simulink model "STEK_roket_simscape_modeli"  (R2025b)
settings: Solver=ode4  StartTime=0.0  StopTime=10.0  FixedStep=0.001  RelTol=1e-3
values from neighbouring files (symbols this model uses):
  m = 0.10*(hi - lo)    [STEK_HIL_grafik_uret.m]
  N = floor(sure_s/TS)    [STEK_HIL_roket_modeli.m]
  s = strrep(sprintf('    [STEK_HIL_grafik_uret.m]
undefined symbols (not defined in the file or in its folder): X, Y, Z
libraries: sm_lib x13, nesl_utility x13, sharedtransform x1
settings Model: SimulationMode=accelerator  Creator=serha  LastModifiedBy=HASAN BARAN

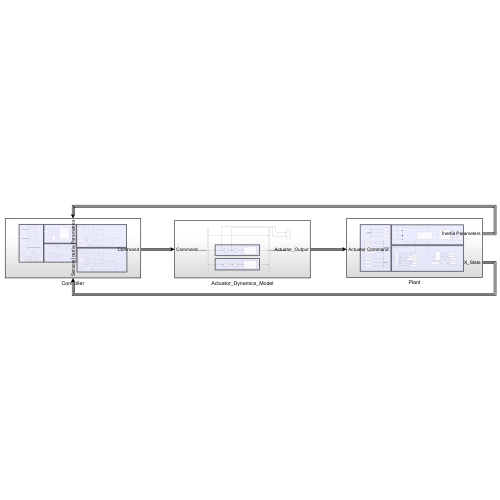
[thumbnail: Simulink's stored preview of the top-level diagram]
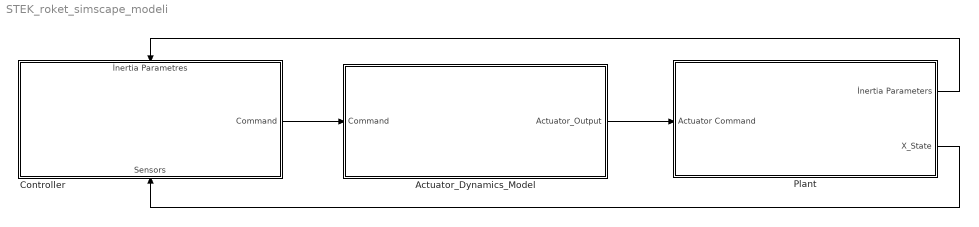
== system STEK_roket_simscape_modeli ==
  Actuator_Dynamics_Model : Subsystem
  Controller : Subsystem
      settings: PortSchema="{\"entries\":[{\"content\":{\"sides\":[{\"content\":{},\"type\":\"ConnectorPlacement.EquallySpacedRectSide\",\"uuid\":\"0baf99d7-4fae-4262-afe2-c6ef4fc7e965\"},{\"content\":{\"connectorIds\":[\"Out1\"],\"side\":\"RIGHT\"},\"type\":\"ConnectorPlacement.EquallySpacedRectSide\",\"uuid\":\"2488a78a-ff3f-460a-aef8-3b0169e54eb5\"},{\"content\":{\"connectorIds\":[\"In1\"],\"side\":\"TOP\"},\"type\":\"ConnectorPlacement.EquallySpacedRectSide\",\"uuid\":\"c1609aa8-bb76-4067-9b78-102063cdf61a\"},{\"content\":{\"connectorIds\":[\"In2\"],\"side\":\"BOTTOM\"},\"type\":\"ConnectorPlacement.EquallySpacedRectSide\",\"uuid\":\"c0f1c736-44b8-4377-a1aa-bd9fc4d2b5f4\"}]},\"type\":\"ConnectorPlacement.EquallySpacedConnector\",\"uuid\":\"1a76828c-b03e-4c12-a774-153e83589147\"}],\"packageUris\":[\"http://schema.mathworks.com/mf0/Connector/R2020b\"],\"version\":\"1.0\"}"
  Plant : Subsystem
  wires:
  Actuator_Dynamics_Model/1(Actuator_Output) -> Plant/1(Actuator Command)
  Controller/1(Command) -> Actuator_Dynamics_Model/1(Command)
  Plant/2(X_State) -> Controller/2(Sensors)
  Plant/1(İnertia Parameters) -> Controller/1(İnertia Parametres)

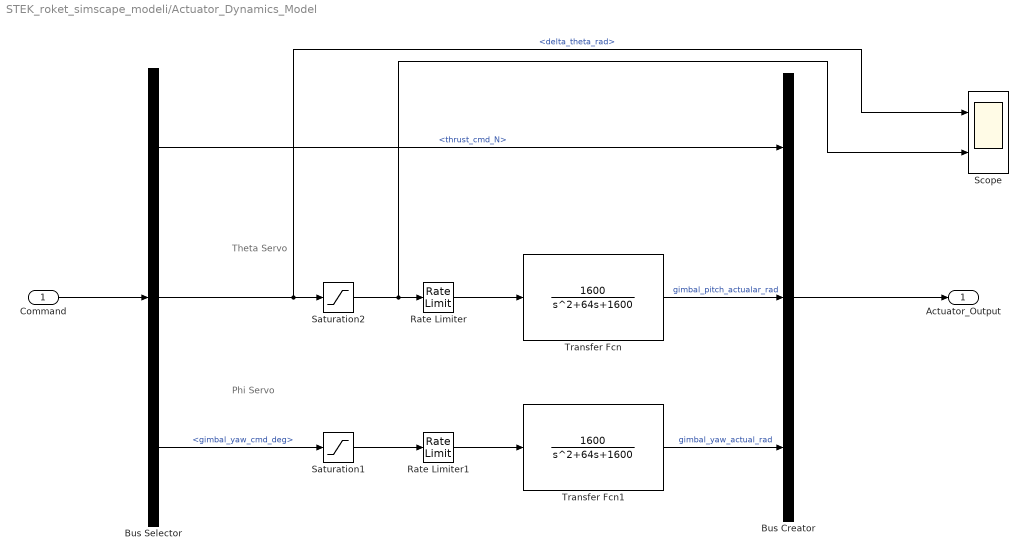
== system STEK_roket_simscape_modeli/Actuator_Dynamics_Model ==
  note: Theta Servo
  note: Phi Servo
  Command : Inport
  Bus Creator : BusCreator  Inputs=3
  Bus Selector : BusSelector  OutputSignals=thrust_cmd_N,delta_theta_rad,gimbal_yaw_cmd_deg
  Rate Limiter : RateLimiter  RisingSlewLimit=428.5  FallingSlewLimit=-428.5  SampleTimeMode=inherited
  Rate Limiter1 : RateLimiter  RisingSlewLimit=428.5  FallingSlewLimit=-428.5  SampleTimeMode=inherited
  Saturation1 : Saturate  UpperLimit=deg2rad(5)  LowerLimit=-deg2rad(5)
  Saturation2 : Saturate  UpperLimit=deg2rad(5)  LowerLimit=-deg2rad(5)
  Scope : Scope  NumInputPorts=2
  Transfer Fcn : TransferFcn  Numerator=1600  Denominator=[1 64 1600]
  Transfer Fcn1 : TransferFcn  Numerator=1600  Denominator=[1 64 1600]
  Actuator_Output : Outport
  wires:
  Command/1 -> Bus Selector/1
  Transfer Fcn/1 -> Bus Creator/2  "gimbal_pitch_actualar_rad"
  Rate Limiter/1 -> Transfer Fcn/1
  Saturation1/1 -> Rate Limiter1/1
  Rate Limiter1/1 -> Transfer Fcn1/1
  Transfer Fcn1/1 -> Bus Creator/3  "gimbal_yaw_actual_rad"
  Bus Selector/3 -> Saturation1/1  "<gimbal_yaw_cmd_deg>"
  Bus Creator/1 -> Actuator_Output/1
  Bus Selector/1 -> Bus Creator/1  "<thrust_cmd_N>"
  Bus Selector/2 -> Scope/1, Saturation2/1  "<delta_theta_rad>"
  Saturation2/1 -> Scope/2, Rate Limiter/1

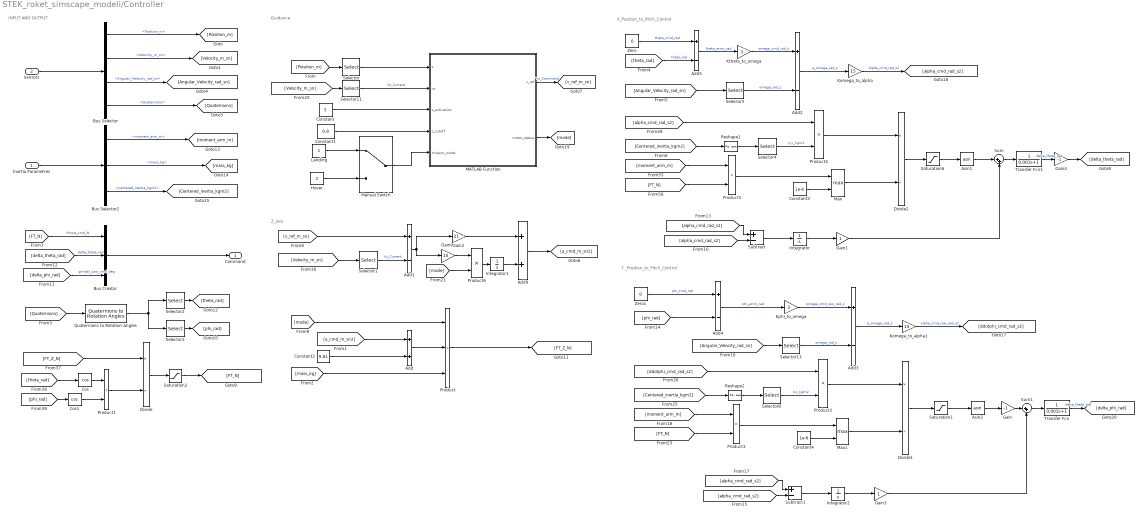
== system STEK_roket_simscape_modeli/Controller ==
  note: Guidance
  note: X_Position_to_Pitch_Control
  note: Z_axis
  note: İNPUT AND OUTPUT
  note: Y _Position_to_Pitch_Control
  İnertia Parametres : Inport
  Sensors : Inport  Port=2
  Add : Sum
  Add{1..5} (5 alike) : Sum  Inputs=+-
  Add9 : Sum
  Asin1 : Trigonometry  Operator=asin
  Asin2 : Trigonometry  Operator=asin
  Bus Creator : BusCreator  Inputs=3
  Bus Selector : BusSelector  OutputSignals=Position_m,Velocity_m_sn,Angular_Velocity_rad_sn,Quaternions
  Bus Selector2 : BusSelector  OutputSignals=moment_arm_m,mass_kg,centered_inertia_kgm2
  Constant : Constant  Value=5
  Constant1 : Constant  Value=0.8
  Constant2 : Constant  Value=9.81
  Constant3 : Constant  Value=1e-6
  Constant4 : Constant  Value=1e-6
  Cos : Trigonometry  Operator=cos
  Cos1 : Trigonometry  Operator=cos
  Divide : Product  Inputs=*/
  Divide1 : Product  Inputs=*/
  Divide2 : Product  Inputs=*/
  Gain : Gain  Gain=-1
  Gain1 : Gain
  Gain2 : Gain  Gain=21
  Gain3 : Gain
  Gain4 : Gain  Gain=-1
  Gain9 : Gain  Gain=15
  Hover : Constant  Value=2
  Integrator : Integrator  LimitOutput=on  UpperSaturationLimit=5  LowerSaturationLimit=-5
  Integrator1 : Integrator  LimitOutput=on  UpperSaturationLimit=7.5  LowerSaturationLimit=-7.5
  Integrator2 : Integrator  LimitOutput=on  UpperSaturationLimit=5  LowerSaturationLimit=-5
  Komega_to_alpha : Gain  Gain=15
  Komega_to_alpha1 : Gain  Gain=15
  Kphi_to_omega : Gain  Gain=3
  Ktheta_to_omega : Gain  Gain=3
  Landing : Constant
  MATLAB Function : MATLAB Function  TreatAsAtomicUnit=on
  Manual Switch : ManualSwitch
  Max : MinMax  Function=max  Inputs=2
  Max1 : MinMax  Function=max  Inputs=2
  Product : Product  Inputs=3
  Product{1..6} (6 alike) : Product
  Quaternions to Rotation Angles : sharedtransform/Quaternions to Rotation Angles  rotationOrder=ZYX  aMode=aMode
  Reshape1 : Reshape
  Reshape2 : Reshape
  Saturation1 : Saturate  UpperLimit=1  LowerLimit=-1
  Saturation2 : Saturate  UpperLimit=600  LowerLimit=0
  Saturation6 : Saturate  UpperLimit=1  LowerLimit=-1
  Selector{,1,3,11,13} (5 alike) : Selector  InputPortWidth=3  IndexOptions=Index vector (dialog)  Indices=3  OutputSizes=1
  Selector2 : Selector  InputPortWidth=3  IndexOptions=Index vector (dialog)  Indices=2  OutputSizes=1
  Selector4 : Selector  InputPortWidth=9  IndexOptions=Index vector (dialog)  Indices=5  OutputSizes=1
  Selector5 : Selector  InputPortWidth=3  IndexOptions=Index vector (dialog)  Indices=2  OutputSizes=1
  Selector8 : Selector  InputPortWidth=9  IndexOptions=Index vector (dialog)  Indices=1  OutputSizes=1
  Subtract : Sum  Inputs=+-
  Subtract1 : Sum  Inputs=+-
  Sum : Sum  Inputs=|++
  Sum1 : Sum  Inputs=|++
  Transfer Fcn : TransferFcn  Denominator=[0.001 1]
  Transfer Fcn1 : TransferFcn  Denominator=[0.001 1]
  Zero : Constant  Value=0  OutDataTypeStr=Inherit: Inherit via back propagation
  Zero1 : Constant  Value=0  OutDataTypeStr=Inherit: Inherit via back propagation
  Command : Outport
  wires:
  Sensors/1 -> Bus Selector/1
  Bus Selector2/2 -> [mass_kg]  "<mass_kg>"
  İnertia Parametres/1 -> Bus Selector2/1
  Bus Selector2/1 -> [moment_arm_m]  "<moment_arm_m>"
  Bus Selector2/3 -> [Centered_inertia_kgm2]  "<centered_inertia_kgm2>"
  Bus Creator/1 -> Command/1
  [delta_phi_rad] -> Bus Creator/3  "gimbal_yaw_cmd_deg"
  [FT_N] -> Bus Creator/1  "thrust_cmd_N"
  [delta_theta_rad] -> Bus Creator/2  "delta_theta_rad"
  [Velocity_m_sn] -> Selector1/1
  Gain2/1 -> Add9/1
  Add1/1 -> Gain9/1, Gain2/1
  Integrator1/1 -> Add9/2
  Selector1/1 -> Add1/2  "Vz_Current"
  Constant2/1 -> Add/2
  [a_cmd_m_sn2] -> Add/1
  Add/1 -> Product/2
  [mass_kg] -> Product/3
  Product/1 -> [FT_Z_N]
  Reshape1/1 -> Selector4/1
  Add5/1 -> Ktheta_to_omega/1  "theta_error_rad"
  Divide2/1 -> Saturation6/1
  [Centered_inertia_kgm2] -> Reshape1/1
  Selector4/1 -> Product4/2  "Iyy_kgm2"
  Sum/1 -> Transfer Fcn1/1
  Product4/1 -> Divide2/1
  Transfer Fcn1/1 -> Gain4/1  "delta_theta_rad"
  Asin1/1 -> Sum/1
  Product5/1 -> Max/1
  [alpha_cmd_rad_s2] -> Product4/1
  [moment_arm_m] -> Product5/1
  [FT_N] -> Product5/2
  Add2/1 -> Komega_to_alpha/1  "e_omega_rad_s"
  Ktheta_to_omega/1 -> Add2/1  "omega_cmd_rad_s"
  [Quaternions] -> Quaternions to Rotation Angles/1
  Quaternions to Rotation Angles/1 -> Selector3/1, Selector2/1
  Selector3/1 -> [phi_rad]
  Selector2/1 -> [theta_rad]
  [Angular_Velocity_rad_sn] -> Selector5/1
  Product1/1 -> Divide/2
  [FT_Z_N] -> Divide/1
  Divide/1 -> Saturation2/1
  Cos1/1 -> Product1/2
  Cos/1 -> Product1/1
  [phi_rad] -> Cos1/1
  [theta_rad] -> Cos/1
  [theta_rad] -> Add5/2  "theta_rad"
  Selector5/1 -> Add2/2  "omega_rad_s"
  [v_ref_m_sn] -> Add1/1
  [mode] -> Product/1
  Max/1 -> Divide2/2
  Constant3/1 -> Max/2
  Saturation6/1 -> Asin1/1
  [mode] -> Product6/2
  Add9/1 -> [a_cmd_m_sn2]
  Gain9/1 -> Product6/1
  Komega_to_alpha/1 -> [alpha_cmd_rad_s2]  "alpha_cmd_rad_s2"
  Saturation1/1 -> Asin2/1
  Constant4/1 -> Max1/2
  Max1/1 -> Divide1/2
  Selector13/1 -> Add3/2  "omega_rad_s"
  [phi_rad] -> Add4/2
  [Angular_Velocity_rad_sn] -> Selector13/1
  Komega_to_alpha1/1 -> [ddotphi_cmd_rad_s2]  "alpha_cmd_raw_rad_s2"
  Kphi_to_omega/1 -> Add3/1  "omega_cmd_raw_rad_s"
  Add3/1 -> Komega_to_alpha1/1  "e_omega_rad_s"
  [FT_N] -> Product3/2
  [moment_arm_m] -> Product3/1
  [ddotphi_cmd_rad_s2] -> Product2/1
  Product3/1 -> Max1/1
  Transfer Fcn/1 -> [delta_phi_rad]  "delta_theta_rad"
  Product2/1 -> Divide1/1
  Selector8/1 -> Product2/2  "Ixx_kgm2"
  [Centered_inertia_kgm2] -> Reshape2/1
  Divide1/1 -> Saturation1/1
  Add4/1 -> Kphi_to_omega/1  "phi_error_rad"
  Reshape2/1 -> Selector8/1
  Asin2/1 -> Gain/1
  Zero/1 -> Add5/1  "theta_cmd_rad"
  Zero1/1 -> Add4/1  "phi_cmd_rad"
  Gain/1 -> Sum1/1
  Bus Selector/3 -> [Angular_Velocity_rad_sn]  "<Angular_Velocity_rad_sn>"
  Bus Selector/2 -> [Velocity_m_sn]  "<Velocity_m_sn>"
  Bus Selector/4 -> [Quaternions]  "<Quaternions>"
  Bus Selector/1 -> [Poisition_m]  "<Position_m>"
  Constant/1 -> MATLAB Function/3(z_activation)
  MATLAB Function/2(motor_status) -> [mode]
  [Poisition_m] -> Selector/1
  Constant1/1 -> MATLAB Function/4(z_cutoff)
  Selector/1 -> MATLAB Function/1(z)
  Selector11/1 -> MATLAB Function/2(vz)  "Vz_Current"
  MATLAB Function/1(v_ref) -> [v_ref_m_sn]  "Vz_Command"
  [Velocity_m_sn] -> Selector11/1
  Saturation2/1 -> [FT_N]
  Product6/1 -> Integrator1/1
  Manual Switch/1 -> MATLAB Function/5(mission_mode)
  Hover/1 -> Manual Switch/2
  Landing/1 -> Manual Switch/1
  [alpha_cmd_rad_s2] -> Subtract/1
  Integrator/1 -> Gain1/1
  Subtract/1 -> Integrator/1
  [alpha_cmd_rad_s2] -> Subtract/2
  Gain1/1 -> Sum/2
  [alpha_cmd_rad_s2] -> Subtract1/2
  Integrator2/1 -> Gain3/1
  Gain3/1 -> Sum1/2
  Subtract1/1 -> Integrator2/1
  [alpha_cmd_rad_s2] -> Subtract1/1
  Sum1/1 -> Transfer Fcn/1
  Gain4/1 -> [delta_theta_rad]

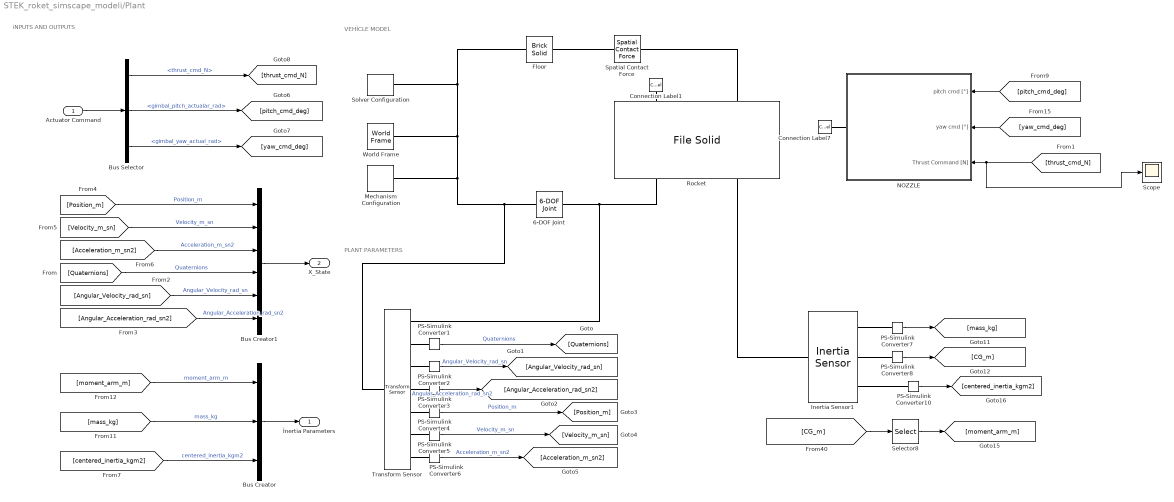
== system STEK_roket_simscape_modeli/Plant ==
  note: VEHİCLE MODEL
  note: iNPUTS AND OUTPUTS
  note: PLANT PARAMETERS
  Actuator Command : Inport
  6-DOF Joint : sm_lib/Joints/6-DOF Joint  JointMode=Normal  CompositeWrenchDir=FollowerOnBase  CompositeWrenchFrame=BaseFrame  SenseConstraintForce=off  SenseConstraintTorque=off  SenseTotalForce=off  SenseTotalTorque=off  PxPositionTargetSpecify=off  PxPositionTargetPriority=High  PxPositionTargetValue=0  PxPositionTargetValueUnits=m  PxVelocityTargetSpecify=off  PxVelocityTargetPriority=High  PxVelocityTargetValue=0  PxVelocityTargetValueUnits=m/s  PxEquilibriumPosition=0  PxEquilibriumPositionUnits=m  PxSpringStiffness=0  PxSpringStiffnessUnits=N/m  PxDampingCoefficient=0  PxDampingCoefficientUnits=N/(m/s)  PxLowerLimitSpecify=off  PxLowerLimitBound=-1  PxLowerLimitBoundUnits=m  PxLowerLimitStiffness=1e6  PxLowerLimitStiffnessUnits=N/m  PxLowerLimitDamping=1e3  PxLowerLimitDampingUnits=N/(m/s)  PxLowerLimitTransitionRegionWidth=1e-4  PxLowerLimitTransitionRegionWidthUnits=m  PxUpperLimitSpecify=off  PxUpperLimitBound=1  PxUpperLimitBoundUnits=m  PxUpperLimitStiffness=1e6  PxUpperLimitStiffnessUnits=N/m  PxUpperLimitDamping=1e3  PxUpperLimitDampingUnits=N/(m/s)  PxUpperLimitTransitionRegionWidth=1e-4  PxUpperLimitTransitionRegionWidthUnits=m  PxTorqueActuationMode=NoTorque  PxMotionActuationMode=ComputedMotion  PxSensePosition=off  PxSenseVelocity=off  PxSenseAcceleration=off  PxSenseTorqueForce=off  PxSenseLowerLimitTorqueForce=off  PxSenseUpperLimitTorqueForce=off  PyPositionTargetSpecify=off  PyPositionTargetPriority=High  PyPositionTargetValue=0  PyPositionTargetValueUnits=m  PyVelocityTargetSpecify=off  PyVelocityTargetPriority=High  PyVelocityTargetValue=0  PyVelocityTargetValueUnits=m/s  PyEquilibriumPosition=0  PyEquilibriumPositionUnits=m  PySpringStiffness=0  PySpringStiffnessUnits=N/m  PyDampingCoefficient=0  PyDampingCoefficientUnits=N/(m/s)  PyLowerLimitSpecify=off  PyLowerLimitBound=-1  PyLowerLimitBoundUnits=m  PyLowerLimitStiffness=1e6  PyLowerLimitStiffnessUnits=N/m  PyLowerLimitDamping=1e3  PyLowerLimitDampingUnits=N/(m/s)  PyLowerLimitTransitionRegionWidth=1e-4  PyLowerLimitTransitionRegionWidthUnits=m  PyUpperLimitSpecify=off  PyUpperLimitBound=1  PyUpperLimitBoundUnits=m  PyUpperLimitStiffness=1e6  PyUpperLimitStiffnessUnits=N/m  PyUpperLimitDamping=1e3  PyUpperLimitDampingUnits=N/(m/s)  PyUpperLimitTransitionRegionWidth=1e-4  PyUpperLimitTransitionRegionWidthUnits=m  PyTorqueActuationMode=NoTorque  PyMotionActuationMode=ComputedMotion  PySensePosition=off  PySenseVelocity=off  PySenseAcceleration=off  PySenseTorqueForce=off  PySenseLowerLimitTorqueForce=off  PySenseUpperLimitTorqueForce=off  PzPositionTargetSpecify=on  PzPositionTargetPriority=High  PzPositionTargetValue=8  PzPositionTargetValueUnits=m  PzVelocityTargetSpecify=off  PzVelocityTargetPriority=High  PzVelocityTargetValue=0  PzVelocityTargetValueUnits=m/s  PzEquilibriumPosition=0  PzEquilibriumPositionUnits=m  PzSpringStiffness=0  PzSpringStiffnessUnits=N/m  PzDampingCoefficient=0  PzDampingCoefficientUnits=N/(m/s)  PzLowerLimitSpecify=off  PzLowerLimitBound=-1  PzLowerLimitBoundUnits=m  PzLowerLimitStiffness=1e6  PzLowerLimitStiffnessUnits=N/m  PzLowerLimitDamping=1e3  PzLowerLimitDampingUnits=N/(m/s)  PzLowerLimitTransitionRegionWidth=1e-4  PzLowerLimitTransitionRegionWidthUnits=m  PzUpperLimitSpecify=off  PzUpperLimitBound=1  PzUpperLimitBoundUnits=m  PzUpperLimitStiffness=1e6  PzUpperLimitStiffnessUnits=N/m  PzUpperLimitDamping=1e3  PzUpperLimitDampingUnits=N/(m/s)  PzUpperLimitTransitionRegionWidth=1e-4  PzUpperLimitTransitionRegionWidthUnits=m  PzTorqueActuationMode=NoTorque  PzMotionActuationMode=ComputedMotion  PzSensePosition=off  PzSenseVelocity=off  PzSenseAcceleration=off  PzSenseTorqueForce=off  PzSenseLowerLimitTorqueForce=off  PzSenseUpperLimitTorqueForce=off  SphPositionTargetSpecify=off  SphPositionTargetPriority=High  SphPositionTargetRotationMethod=StandardAxis  SphPositionTargetFollAlignAxisA=+X  SphPositionTargetBaseAlignAxisA=+Y  SphPositionTargetFollAlignAxisB=+Y  SphPositionTargetBaseAlignAxisB=+Z  SphPositionTargetRotationStandardAxis=+X  SphPositionTargetRotationAngle=5  SphPositionTargetRotationAngleUnits=deg  SphPositionTargetRotationArbitraryAxis=[0 0 1]  SphPositionTargetRotationSequenceAxes=FollowerAxes  SphPositionTargetRotationSequence=ZYX  SphPositionTargetRotationSequenceAngles=[0 0 0]  SphPositionTargetRotationSequenceAnglesUnits=deg  SphPositionTargetRotationMatrix=[1 0 0;0 1 0;0 0 1]  SphPositionTargetQuaternion=[1 0 0 0]  SphVelocityTargetSpecify=off  SphVelocityTargetPriority=High  SphVelocityTargetValue=[0 0 0]  SphVelocityTargetValueUnits=deg/s  SphVelocityTargetInFollowerFrame=on  SphEqPosRotationMethod=None  SphEqPosFollAlignAxisA=+X  SphEqPosBaseAlignAxisA=+Y  SphEqPosFollAlignAxisB=+Y  SphEqPosBaseAlignAxisB=+Z  SphEqPosRotationStandardAxis=+Z  SphEqPosRotationAngle=0  SphEqPosRotationAngleUnits=deg  SphEqPosRotationArbitraryAxis=[0 0 1]  SphEqPosRotationSequenceAxes=FollowerAxes  SphEqPosRotationSequence=XYX  SphEqPosRotationSequenceAngles=[0 0 0]  SphEqPosRotationSequenceAnglesUnits=deg  SphEqPosRotationMatrix=[1 0 0;0 1 0;0 0 1]  SphEqPosQuaternion=[1 0 0 0]  SphSpringStiffness=0  SphSpringStiffnessUnits=N*m/deg  SphDampingCoefficient=0  SphDampingCoefficientUnits=N*m/(deg/s)  SphLowerLimitSpecify=off  SphLowerLimitBound=15  SphLowerLimitBoundUnits=deg  SphLowerLimitStiffness=1e4  SphLowerLimitStiffnessUnits=N*m/deg  SphLowerLimitDamping=10  SphLowerLimitDampingUnits=N*m/(deg/s)  SphLowerLimitTransitionRegionWidth=0.1  SphLowerLimitTransitionRegionWidthUnits=deg  SphUpperLimitSpecify=off  SphUpperLimitBound=45  SphUpperLimitBoundUnits=deg  SphUpperLimitStiffness=1e4  SphUpperLimitStiffnessUnits=N*m/deg  SphUpperLimitDamping=10  SphUpperLimitDampingUnits=N*m/(deg/s)  SphUpperLimitTransitionRegionWidth=0.1  SphUpperLimitTransitionRegionWidthUnits=deg  SphTorqueActuationMode=NoTorque  SphActuateTorqueX=off  SphActuateTorqueY=off  SphActuateTorqueZ=off  SphActuateTorque=off  SphActuationFrame=BaseFrame  SphSensePosition=off  SphSenseVelocityX=off  SphSenseVelocityY=off  SphSenseVelocityZ=off  SphSenseVelocity=off  SphSenseAccelerationX=off  SphSenseAccelerationY=off  SphSenseAccelerationZ=off  SphSenseAcceleration=off  SphSenseLowerLimitTorqueMag=off  SphSenseUpperLimitTorqueMag=off  SphSensingFrame=BaseFrame
  Bus Creator : BusCreator  Inputs=3
  Bus Creator1 : BusCreator  Inputs=6
  Bus Selector : BusSelector  OutputSignals=thrust_cmd_N,gimbal_pitch_actualar_rad,gimbal_yaw_actual_rad
  Connection Label1 : ConnectionLabel  Label=NOZZLE
  Connection Label7 : ConnectionLabel  Label=NOZZLE
  Floor : sm_lib/Body Elements/Brick Solid  BrickDimensions=[5 5 0.5]  BrickDimensionsUnits=m  ExportEntireGeometry=on  InertiaType=CalculateFromGeometry  BasedOnType=Density  Density=0  DensityUnits=kg/m^3  Mass=1  MassUnits=kg  CenterOfMass=[0 0 0]  CenterOfMassUnits=m  MomentsOfInertia=[1 1 1]  MomentsOfInertiaUnits=kg*m^2  ProductsOfInertia=[0 0 0]  ProductsOfInertiaUnits=kg*m^2  GraphicType=FromGeometry  MarkerShape=Sphere  MarkerSize=10  GraphicVisPropType=SimpleVisualProperties  GraphicDiffuseColor=[1 0.6667 0]  GraphicOpacity=1  GraphicSpecularColor=[0.5 0.5 0.5 1.0]  GraphicAmbientColor=[0.15 0.15 0.15 1.0]  GraphicEmissiveColor=[0.0 0.0 0.0 1.0]  GraphicShininess=75  DoExposeReferenceFrame=on  SerializedFrames=<Frames/>
  Inertia Sensor1 : sm_lib/Body Elements/Inertia Sensor  SensorExtent=Mechanism  SpanWeldJoints=off  ExcludeGroundedBodies=off  MeasurementFrame=Attached  SenseMass=on  SenseCenterOfMass=on  SenseInertiaMatrix=off  SenseCenteredInertiaMatrix=on  SensePrincipalInertiaMatrix=off  SenseRotationMatrix=off  GraphicType=PrincipalInertiaFrame  PrincipalInertiaFrameSize=20  GraphicVisPropType=SimpleVisualProperties  GraphicDiffuseColor=[0.5 0.5 0.5]  GraphicOpacity=1  GraphicSpecularColor=[0.5 0.5 0.5 1.0]  GraphicAmbientColor=[0.15 0.15 0.15 1.0]  GraphicEmissiveColor=[0.0 0.0 0.0 1.0]  GraphicShininess=75
  Mechanism Configuration : sm_lib/Utilities/Mechanism Configuration  UniformGravity=Constant  GravityVector=[0 0 -9.80665]  GravityVectorUnits=m/s^2  LinearizationDelta=0.001  JointModeTransitionNonlinearIterations=2
  NOZZLE : Subsystem
  PS-Simulink Converter{1..8,10} (9 alike) : nesl_utility/PS-Simulink Converter  PhysicalDomain=network_engine_domain  SubClassName=ps_output  LeftPortType=input  RightPortType=output  PseudoPeriodic=off  Frequencies=[]  VectorFormat=inherit  Unit=inherit  AffineConversion=off
  Rocket : sm_lib/Body Elements/File Solid  ExtGeomFileName=C:\Users\HASAN BARAN\Desktop\Stek ahr\AHR CAD DOSYALARI\Tvc yok koordinat.STEP  UnitType=Custom  ExtGeomFileUnits=mm  StepReaderType=HEX  ExportConvexHullGeometry=on  InertiaType=CalculateFromGeometry  BasedOnType=Mass  Density=1000  DensityUnits=kg/m^3  Mass=32  MassUnits=kg  CenterOfMass=[0 0 0]  CenterOfMassUnits=m  MomentsOfInertia=[1 1 1]  MomentsOfInertiaUnits=kg*m^2  ProductsOfInertia=[0 0 0]  ProductsOfInertiaUnits=kg*m^2  GraphicType=FromGeometry  MarkerShape=Sphere  MarkerSize=10  GraphicVisPropType=SimpleVisualProperties  GraphicDiffuseColor=[0.5 0.5 0.5]  GraphicOpacity=1  GraphicSpecularColor=[0.5 0.5 0.5 1.0]  GraphicAmbientColor=[0.15 0.15 0.15 1.0]  GraphicEmissiveColor=[0.0 0.0 0.0 1.0]  GraphicShininess=75  DoExposeReferenceFrame=off  SerializedFrames=<Frames><Frame><Id>Frame1</Id><Value><Name>CoM</Name><Origin><Source>CenterOfMassFrame</Source><FeatureName></FeatureName></Origin><PrimaryAxis><DefinedDirection>+Z</DefinedDirection><Source>ReferenceFrame</Source><SourceDirection>+Z</SourceDirection><FeatureName></FeatureName></PrimaryAxis><SecondaryAxis><DefinedDirection>+X</DefinedDirection><Source>ReferenceFrame</Source><SourceDirection>+X</SourceDirection><FeatureName></FeatureName></SecondaryAxis></Value></Frame><Frame><Id>Frame2</Id><Value><Name>TVC</Name><Origin><Source>GeometricFeature</Source><FeatureName>planar surface 130</FeatureName></Origin><PrimaryAxis><DefinedDirection>+Z</DefinedDirection><Source>ReferenceFrame</Source><SourceDirection>+X</SourceDirection><FeatureName></FeatureName></PrimaryAxis><SecondaryAxis><DefinedDirection>+X</DefinedDirection><Source>ReferenceFrame</Source><SourceDirection>-Z</SourceDirection><FeatureName></FeatureName></SecondaryAxis></Value></Frame><Frame><Id>Frame3</Id><Value><Name>İnertia_Sensor</Name><Origin><Source>GeometricFeature</Source><FeatureName>planar surface 130</FeatureName></Origin><PrimaryAxis><DefinedDirection>+Z</DefinedDirection><Source>ReferenceFrame</Source><SourceDirection>+Z</SourceDirection><FeatureName></FeatureName></PrimaryAxis><SecondaryAxis><DefinedDirection>+X</DefinedDirection><Source>ReferenceFrame</Source><SourceDirection>+X</SourceDirection><FeatureName></FeatureName></SecondaryAxis></Value></Frame></Frames>
  Scope : Scope
      settings: ActiveDisplayYMinimum=-1  ActiveDisplayYMaximum=1
  Selector8 : Selector  InputPortWidth=3  IndexOptions=Index vector (dialog)  Indices=3  OutputSizes=1
  Solver Configuration : nesl_utility/Solver Configuration  PhysicalDomain=network_engine_domain  SubClassName=solver  LeftPortType=input  RightPortType=generic  Tones=[]  Harmonics=[]  SimulateNoise=off  Profile=off  UseLocalSampling=off  EnableSwitchedLinearOptims=on  FrequencyDomain=off  UseCCode=off  RelTol=0.001  AbsTol=1e-06  MinStep=1e-09  ToWorkspace=off  RevertToSquareIcSolve=off  NumHomotopyIterations=100  PhasorMode=off  PhasorModeNumHarmonics=1  ConsistencySolver=NEWTON_XTOL_AFTER_FTOL  IndexReductionMethod=DerivativeReplacement  DoDC=off  ResidualTolerance=1e-09  ConsistencyTolSource=GLOBAL  ConsistencyAbsTol=0.001  ConsistencyRelTol=0.001  ConsistencyTolFactor=0.001  UseLocalSolver=off  LocalSolverChoice=NE_BACKWARD_EULER_ADVANCER  ResolveIndetEquations=on  FunctionEvalNumThread=1  LocalSolverSampleTime=0.001  DoFixedCost=off  MaxNonlinIter=3  MaxModeIter=2  ComputeImpulses=off  ImpulseIterations=2  LinearAlgebra=Sparse  LinearAlgebraNumThread=0  EquationFormulation=NE_TIME_EF  DelaysMemoryBudget=1024  AutomaticFiltering=on  FilteringTimeConstant=0.001  PartitionStorageMethod=AS_NEEDED  PartitionMemoryBudget=1024  PartitionMethod=FAST  MultibodyUseLocalSolver=off  MultibodyLocalSolverChoice=ODE1  MultibodyLocalSolverSampleTime=0.001
  Spatial Contact Force : sm_lib/Forces and Torques/Spatial Contact Force  SenseSeparationDistance=off  NormalForceType=SmoothSpringDamper  NormalStiffness=1e6  NormalStiffnessUnits=N/m  NormalDamping=1e3  NormalDampingUnits=N/(m/s)  NormalTransitionRegionWidth=1e-4  NormalTransitionRegionWidthUnits=m  FrictionType=SmoothStickSlip  CoefficientOfStaticFriction=0.5  CoefficientOfDynamicFriction=0.3  FrictionalCriticalVelocity=1e-3  FrictionalCriticalVelocityUnits=m/s  SenseContactSignal=off  SensePenetrationDepth=off  SenseNormalVelocity=off  SenseTangentialVelocity=off  SensingForceTorqueDirection=BaseOnFollower  SensingForceTorqueResolutionFrame=ContactFrame  SenseNormalForce=off  SenseNormalForceMagnitude=off  SenseNormalTorque=off  SenseFrictionalForce=off  SenseFrictionalForceMagnitude=off  SenseFrictionalTorque=off  SenseTotalForce=off  SenseTotalTorque=off  SenseContactBaseRotation=off  SenseContactBaseTranslation=off  SenseContactFollowerRotation=off  SenseContactFollowerTranslation=off  ZeroCrossDetectContactStartAndEnd=off
  Transform Sensor : sm_lib/Frames and Transforms/Transform Sensor  MeasurementFrame=World  RotationSequence=ZYX  SenseAngle=off  SenseAxis=off  SenseQ=on  SenseR=off  SenseRotationSequence=off  SenseOmegaX=off  SenseOmegaY=off  SenseOmegaZ=off  SenseOmega=on  SenseQDot=off  SenseRDot=off  SenseRotationSequenceDot=off  SenseAlphaX=off  SenseAlphaY=off  SenseAlphaZ=off  SenseAlpha=on  SenseQDDot=off  SenseRDDot=off  SenseX=off  SenseY=off  SenseZ=off  SenseXYZ=on  SenseRad=off  SenseAzim=off  SenseDist=off  SenseInc=off  SenseXDot=off  SenseYDot=off  SenseZDot=off  SenseXYZDot=on  SenseRadDot=off  SenseAzimDot=off  SenseDistDot=off  SenseIncDot=off  SenseXDDot=off  SenseYDDot=off  SenseZDDot=off  SenseXYZDDot=on  SenseRadDDot=off  SenseAzimDDot=off  SenseDistDDot=off  SenseIncDDot=off
  World Frame : sm_lib/Frames and Transforms/World Frame
  İnertia Parameters : Outport
  X_State : Outport  Port=2
  wires:
  Bus Creator1/1 -> X_State/1
  Actuator Command/1 -> Bus Selector/1
  [Position_m] -> Bus Creator1/1  "Position_m"
  PS-Simulink Converter7/1 -> [mass_kg]
  [Quaternions] -> Bus Creator1/4  "Quaternions"
  Bus Selector/3 -> [yaw_cmd_deg]  "<gimbal_yaw_actual_rad>"
  [centered_inertia_kgm2] -> Bus Creator/3  "centered_inertia_kgm2"
  Bus Creator/1 -> İnertia Parameters/1
  [Velocity_m_sn] -> Bus Creator1/2  "Velocity_m_sn"
  PS-Simulink Converter3/1 -> [Angular_Acceleration_rad_sn2]  "Angular_Acceleration_rad_sn2"
  [Angular_Acceleration_rad_sn2] -> Bus Creator1/6  "Angular_Acceleration_rad_sn2"
  [Acceleration_m_sn2] -> Bus Creator1/3  "Acceleration_m_sn2"
  Selector8/1 -> [moment_arm_m]
  PS-Simulink Converter8/1 -> [CG_m]
  [moment_arm_m] -> Bus Creator/1  "moment_arm_m"
  PS-Simulink Converter1/1 -> [Quaternions]  "Quaternions"
  [mass_kg] -> Bus Creator/2  "mass_kg"
  [CG_m] -> Selector8/1
  PS-Simulink Converter6/1 -> [Acceleration_m_sn2]  "Acceleration_m_sn2"
  PS-Simulink Converter5/1 -> [Velocity_m_sn]  "Velocity_m_sn"
  PS-Simulink Converter2/1 -> [Angular_Velocity_rad_sn]  "Angular_Velocity_rad_sn"
  Bus Selector/2 -> [pitch_cmd_deg]  "<gimbal_pitch_actualar_rad>"
  PS-Simulink Converter10/1 -> [centered_inertia_kgm2]
  PS-Simulink Converter4/1 -> [Position_m]  "Position_m"
  [Angular_Velocity_rad_sn] -> Bus Creator1/5  "Angular_Velocity_rad_sn"
  [yaw_cmd_deg] -> NOZZLE/2(yaw cmd [°])
  [pitch_cmd_deg] -> NOZZLE/1(pitch cmd [°])
  [thrust_cmd_N] -> Scope/1, NOZZLE/3(Thrust Command [N])
  Bus Selector/1 -> [thrust_cmd_N]  "<thrust_cmd_N>"
  connections:
  World Frame/RConn1 -- Floor/RConn1 -- Solver Configuration/RConn1 -- Transform Sensor/LConn1 -- 6-DOF Joint/LConn1 -- Mechanism Configuration/RConn1
  Rocket/LConn1 -- 6-DOF Joint/RConn1 -- Transform Sensor/RConn1
  Connection Label1/LConn1 -- Rocket/RConn1
  Floor/LConn1 -- Spatial Contact Force/LConn1
  Inertia Sensor1/RConn3 -- PS-Simulink Converter10/LConn1
  NOZZLE/RConn1 -- Connection Label7/LConn1
  Transform Sensor/RConn6 -- PS-Simulink Converter5/LConn1
  PS-Simulink Converter7/LConn1 -- Inertia Sensor1/RConn1
  Transform Sensor/RConn7 -- PS-Simulink Converter6/LConn1
  PS-Simulink Converter3/LConn1 -- Transform Sensor/RConn4
  Rocket/RConn2 -- Spatial Contact Force/RConn1
  PS-Simulink Converter4/LConn1 -- Transform Sensor/RConn5
  PS-Simulink Converter1/LConn1 -- Transform Sensor/RConn2
  PS-Simulink Converter2/LConn1 -- Transform Sensor/RConn3
  Inertia Sensor1/RConn2 -- PS-Simulink Converter8/LConn1
  Rocket/LConn2 -- Inertia Sensor1/LConn1

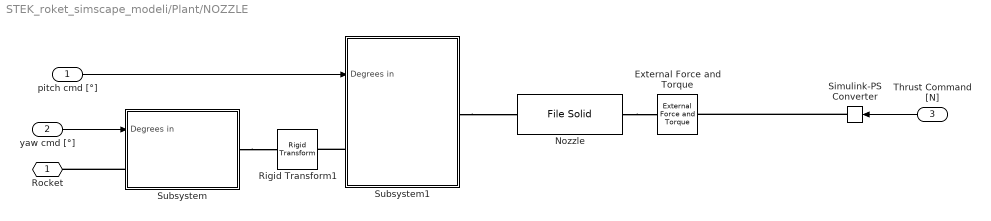
== system STEK_roket_simscape_modeli/Plant/NOZZLE ==
  pitch cmd [°] : Inport
  yaw cmd [°] : Inport  Port=2
  Thrust Command [N] : Inport  Port=3
  External Force and Torque : sm_lib/Forces and Torques/External Force and Torque  EnableForceX=off  EnableForceY=off  EnableForceZ=on  EnableForce=off  ForceResolutionFrame=AttachedFrame  EnableTorqueX=off  EnableTorqueY=off  EnableTorqueZ=off  EnableTorque=off  TorqueResolutionFrame=AttachedFrame
  Nozzle : sm_lib/Body Elements/File Solid  ExtGeomFileName=C:\Users\HASAN BARAN\Desktop\Stek ahr\AHR CAD DOSYALARI\Tvc montaj koordinat.STEP  UnitType=FromFile  ExtGeomFileUnits=m  StepReaderType=HEX  ExportConvexHullGeometry=off  InertiaType=CalculateFromGeometry  BasedOnType=Mass  Density=1000  DensityUnits=kg/m^3  Mass=1.8  MassUnits=kg  CenterOfMass=[0 0 0]  CenterOfMassUnits=m  MomentsOfInertia=[1 1 1]  MomentsOfInertiaUnits=kg*m^2  ProductsOfInertia=[0 0 0]  ProductsOfInertiaUnits=kg*m^2  GraphicType=FromGeometry  MarkerShape=Sphere  MarkerSize=10  GraphicVisPropType=SimpleVisualProperties  GraphicDiffuseColor=[0.5 0.5 0.5]  GraphicOpacity=1  GraphicSpecularColor=[0.5 0.5 0.5 1.0]  GraphicAmbientColor=[0.15 0.15 0.15 1.0]  GraphicEmissiveColor=[0.0 0.0 0.0 1.0]  GraphicShininess=75  DoExposeReferenceFrame=off  SerializedFrames=<Frames><Frame><Id>Frame1</Id><Value><Name>Rocket</Name><Origin><Source>GeometricFeature</Source><FeatureName>planar surface 43</FeatureName></Origin><PrimaryAxis><DefinedDirection>+Z</DefinedDirection><Source>ReferenceFrame</Source><SourceDirection>+Y</SourceDirection><FeatureName></FeatureName></PrimaryAxis><SecondaryAxis><DefinedDirection>-Y</DefinedDirection><Source>ReferenceFrame</Source><SourceDirection>+X</SourceDirection><FeatureName></FeatureName></SecondaryAxis></Value></Frame><Frame><Id>Frame2</Id><Value><Name>Thrust</Name><Origin><Source>GeometricFeature</Source><FeatureName>planar surface 44</FeatureName></Origin><PrimaryAxis><DefinedDirection>+Z</DefinedDirection><Source>ReferenceFrame</Source><SourceDirection>+Z</SourceDirection><FeatureName></FeatureName></PrimaryAxis><SecondaryAxis><DefinedDirection>+X</DefinedDirection><Source>ReferenceFrame</Source><SourceDirection>+X</SourceDirection><FeatureName></FeatureName></SecondaryAxis></Value></Frame></Frames>
  Rigid Transform1 : sm_lib/Frames and Transforms/Rigid Transform  RotationMethod=StandardAxis  FollAlignAxisA=+X  BaseAlignAxisA=+Y  FollAlignAxisB=+Y  BaseAlignAxisB=+Z  RotationStandardAxis=+X  RotationAngle=-90  RotationAngleUnits=deg  RotationArbitraryAxis=[0 0 1]  RotationSequenceAxes=FollowerAxes  RotationSequence=XYX  RotationSequenceAngles=[0 0 0]  RotationSequenceAnglesUnits=deg  RotationMatrix=[1 0 0;0 1 0;0 0 1]  Quaternion=[1 0 0 0]  TranslationMethod=None  TranslationCartesianOffset=[0 0 0]  TranslationCartesianOffsetUnits=m  TranslationStandardAxis=+Z  TranslationStandardOffset=0  TranslationStandardOffsetUnits=m  TranslationROffset=0  TranslationROffsetUnits=m  TranslationThetaOffset=0  TranslationThetaOffsetUnits=deg  TranslationZOffset=0  TranslationZOffsetUnits=m
  Simulink-PS Converter : nesl_utility/Simulink-PS Converter  PhysicalDomain=network_engine_domain  SubClassName=ps_input  LeftPortType=input  RightPortType=output  PseudoPeriodic=off  Frequencies=[]  NoiseDistribution=none  NoiseParameters=[]  Unit=1  AffineConversion=off  FilteringAndDerivatives=provide  SimscapeFilterOrder=1  InputFilterTimeConstant=0.001  UdotUserProvided=0
  Subsystem : Subsystem
  Subsystem1 : Subsystem
  Rocket : PMIOPort  Side=Right
  wires:
  yaw cmd [°]/1 -> Subsystem/1(Degrees in)
  Thrust Command [N]/1 -> Simulink-PS Converter/1
  pitch cmd [°]/1 -> Subsystem1/1(Degrees in)
  connections:
  Subsystem/RConn1 -- Rigid Transform1/LConn1
  Subsystem1/LConn1 -- Rigid Transform1/RConn1
  Subsystem/LConn1 -- Rocket/RConn1
  Nozzle/RConn1 -- External Force and Torque/RConn1
  Simulink-PS Converter/RConn1 -- External Force and Torque/LConn1
  Subsystem1/RConn1 -- Nozzle/LConn1

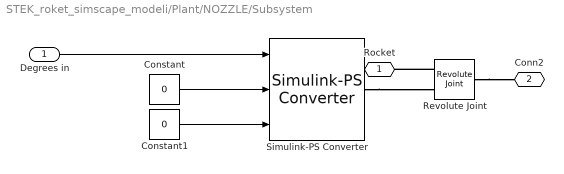
== system STEK_roket_simscape_modeli/Plant/NOZZLE/Subsystem ==
  Degrees in : Inport
  Constant : Constant  Value=0
  Constant1 : Constant  Value=0
  Revolute Joint : sm_lib/Joints/Revolute Joint  JointMode=Normal  CompositeWrenchDir=FollowerOnBase  CompositeWrenchFrame=BaseFrame  SenseConstraintForce=off  SenseConstraintTorque=off  SenseTotalForce=off  SenseTotalTorque=off  PositionTargetSpecify=off  PositionTargetPriority=High  PositionTargetValue=0  PositionTargetValueUnits=deg  VelocityTargetSpecify=off  VelocityTargetPriority=High  VelocityTargetValue=0  VelocityTargetValueUnits=deg/s  EquilibriumPosition=0  EquilibriumPositionUnits=deg  SpringStiffness=0  SpringStiffnessUnits=N*m/deg  DampingCoefficient=0  DampingCoefficientUnits=N*m/(deg/s)  LowerLimitSpecify=off  LowerLimitBound=-90  LowerLimitBoundUnits=deg  LowerLimitStiffness=1e4  LowerLimitStiffnessUnits=N*m/deg  LowerLimitDamping=10  LowerLimitDampingUnits=N*m/(deg/s)  LowerLimitTransitionRegionWidth=0.1  LowerLimitTransitionRegionWidthUnits=deg  UpperLimitSpecify=off  UpperLimitBound=90  UpperLimitBoundUnits=deg  UpperLimitStiffness=1e4  UpperLimitStiffnessUnits=N*m/deg  UpperLimitDamping=10  UpperLimitDampingUnits=N*m/(deg/s)  UpperLimitTransitionRegionWidth=0.1  UpperLimitTransitionRegionWidthUnits=deg  TorqueActuationMode=ComputedTorque  MotionActuationMode=InputMotion  SensePosition=off  SenseVelocity=off  SenseAcceleration=off  SenseTorqueForce=off  SenseLowerLimitTorqueForce=off  SenseUpperLimitTorqueForce=off
  Simulink-PS Converter : nesl_utility/Simulink-PS Converter  PhysicalDomain=network_engine_domain  SubClassName=ps_input  LeftPortType=input  RightPortType=output  PseudoPeriodic=off  Frequencies=[]  NoiseDistribution=none  NoiseParameters=[]  Unit=1  AffineConversion=off  FilteringAndDerivatives=provide  SimscapeFilterOrder=1  InputFilterTimeConstant=0.001  UdotUserProvided=2
  Rocket : PMIOPort  Side=Left
  Conn2 : PMIOPort  Port=2  Side=Right
  wires:
  Constant/1 -> Simulink-PS Converter/2
  Degrees in/1 -> Simulink-PS Converter/1
  Constant1/1 -> Simulink-PS Converter/3
  connections:
  Revolute Joint/RConn1 -- Conn2/RConn1
  Revolute Joint/LConn1 -- Rocket/RConn1
  Simulink-PS Converter/RConn1 -- Revolute Joint/LConn2

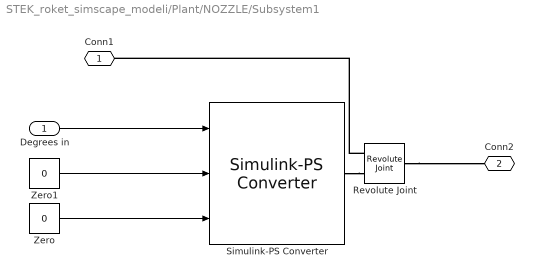
== system STEK_roket_simscape_modeli/Plant/NOZZLE/Subsystem1 ==
  Degrees in : Inport
  Revolute Joint : sm_lib/Joints/Revolute Joint  JointMode=Normal  CompositeWrenchDir=FollowerOnBase  CompositeWrenchFrame=BaseFrame  SenseConstraintForce=off  SenseConstraintTorque=off  SenseTotalForce=off  SenseTotalTorque=off  PositionTargetSpecify=off  PositionTargetPriority=High  PositionTargetValue=0  PositionTargetValueUnits=deg  VelocityTargetSpecify=off  VelocityTargetPriority=High  VelocityTargetValue=0  VelocityTargetValueUnits=deg/s  EquilibriumPosition=0  EquilibriumPositionUnits=deg  SpringStiffness=0  SpringStiffnessUnits=N*m/deg  DampingCoefficient=0  DampingCoefficientUnits=N*m/(deg/s)  LowerLimitSpecify=off  LowerLimitBound=-90  LowerLimitBoundUnits=deg  LowerLimitStiffness=1e4  LowerLimitStiffnessUnits=N*m/deg  LowerLimitDamping=10  LowerLimitDampingUnits=N*m/(deg/s)  LowerLimitTransitionRegionWidth=0.1  LowerLimitTransitionRegionWidthUnits=deg  UpperLimitSpecify=off  UpperLimitBound=90  UpperLimitBoundUnits=deg  UpperLimitStiffness=1e4  UpperLimitStiffnessUnits=N*m/deg  UpperLimitDamping=10  UpperLimitDampingUnits=N*m/(deg/s)  UpperLimitTransitionRegionWidth=0.1  UpperLimitTransitionRegionWidthUnits=deg  TorqueActuationMode=ComputedTorque  MotionActuationMode=InputMotion  SensePosition=off  SenseVelocity=off  SenseAcceleration=off  SenseTorqueForce=off  SenseLowerLimitTorqueForce=off  SenseUpperLimitTorqueForce=off
  Simulink-PS Converter : nesl_utility/Simulink-PS Converter  PhysicalDomain=network_engine_domain  SubClassName=ps_input  LeftPortType=input  RightPortType=output  PseudoPeriodic=off  Frequencies=[]  NoiseDistribution=none  NoiseParameters=[]  Unit=1  AffineConversion=off  FilteringAndDerivatives=provide  SimscapeFilterOrder=1  InputFilterTimeConstant=0.001  UdotUserProvided=2
  Zero : Constant  Value=0  OutDataTypeStr=Inherit: Inherit via back propagation
  Zero1 : Constant  Value=0  OutDataTypeStr=Inherit: Inherit via back propagation
  Conn1 : PMIOPort  Side=Left
  Conn2 : PMIOPort  Port=2  Side=Right
  wires:
  Zero/1 -> Simulink-PS Converter/3
  Zero1/1 -> Simulink-PS Converter/2
  Degrees in/1 -> Simulink-PS Converter/1
  connections:
  Simulink-PS Converter/RConn1 -- Revolute Joint/LConn2
  Revolute Joint/LConn1 -- Conn1/RConn1
  Revolute Joint/RConn1 -- Conn2/RConn1

== matlab function STEK_roket_simscape_modeli/Controller/MATLAB Function ==
  settings: updateMethod=DISCRETE
  data: z input; vz input; v_ref output; z_activation input; z_cutoff input; motor_status output; mission_mode input
function [v_ref, motor_status] = landing_logic(z, vz, z_activation, z_cutoff, mission_mode)
%#codegen
% z             : İrtifa [m], + yukarı
% vz            : Düşey hız [m/s], + yukarı, - aşağı (Düşerken negatiftir)
% z_activation  : Aktivasyon irtifası (Burası artık kesinlikle 5.0)
% z_cutoff      : İtki kesme irtifası [m] (Örn: 0.08)
% mission_mode  : 1 = Landing Modu, 2 = Hover Modu, Diğer = Motor Kapalı

% Kalıcı (Persistent) Değişken: Sistem ilk açıldığında serbest düşüş hızını kilitlemek için
persistent v_entry_speed;
if isempty(v_entry_speed)
    v_entry_speed = -8.86; % Teorik başlangıç tahmini (9 metreden düşen 33 kg için)
end

% Negatif irtifa koruması
if z < 0.0
    z = 0.0;
end

% =========================================================
% YENİ AGRESİF PARAMETRELER (5 METRE SERBEST DÜŞÜŞ SENARYOSU)
% =========================================================
z_flare_start = 4.90;       % [m] Sistem açılır açılmaz (5m) frenleme başlasın diye pay
z_touch_zone  = 0.25;       % [m] Son dokunuş bölgesi yüksekliği
v_land_touch  = -0.15;      % [m/s] Hedeflenen güvenli temas hızı (Max 0.20'nin altında)
vz_cutoff_min = -0.25;      % [m/s] Motor kesme için maksimum dikey hız
vz_cutoff_max =  0.05;      % [m/s] Motor kesme için minimum dikey hız

% =========================================================
% HOVER BÖLGESİ PARAMETRELERİ (MISSION_MODE == 2)
% =========================================================
z_hover_target = 5.0;       % [m] Hedeflenen hover yüksekliği
z_hover_start  = 2.0;       % [m] Hover modunun başladığı zemin yüksekliği
v_climb        = 0.50;      % [m/s] Güvenli tırmanış hızı referansı (Pozitif)

% =========================================================
% ANA MANTIĞIN ÇALIŞTIRILMASI
% =========================================================
if mission_mode == 1
    % LANDING MODU
    if z > z_activation
        % 5 metrenin üstündeyiz: Tam serbest düşüş, motorlar kapalı
        v_ref = 0.0;
        motor_status = 0.0;
        v_entry_speed = vz; % Sistem devreye girene kadar anlık hızı hafızada tut
        
    elseif (z <= z_cutoff) && (vz >= vz_cutoff_min) && (vz <= vz_cutoff_max)
        % Yere ulaşıldı ve hız güvenli sınırda: Motorları tamamen kapat
        v_ref = 0.0;
        motor_status = 0.0;
        
    else
        % AKTİF ACİL FRENLEME BÖLGESİ (z <= 5m)
        motor_status = 1.0; % Motorlar hemen aktif!
        
        if z > z_flare_start
            % Tetiklenmenin ilk saliseleri için referansı giriş hızına eşitle
            v_cmd = v_entry_speed;
            
        elseif z > z_touch_zone
            % Dinamik Rampalama:
            % Araç 5 metreden girdikten sonra hızı v_entry_speed'den v_land_touch'a lineer düşürür
            denom = z_flare_start - z_touch_zone;
            if denom < 1e-4, denom = 1e-4; end
            
            ratio = (z - z_touch_zone) / denom;
            ratio = max(min(ratio, 1.0), 0.0); % 0 ile 1 arasına sıkıştır
            
            % Frenleme referans hızı hesabı
            v_cmd = v_land_touch + ratio * (v_entry_speed - v_land_touch);
        else
            % Son 25 cm: Hedeflenen 0.15 m/s hızla yumuşak dokunuş yap
            v_cmd = v_land_touch;
        end
        
        v_ref = v_cmd;
    end
    
elseif mission_mode == 2
    % =========================================================
    % HOVER MODU EKLENTİSİ
    % =========================================================
    motor_status = 1.0; % Motorlar hover için kesinlikle aktif olmalı
    
    if z >= z_hover_target
        % Araç 5 metreye ulaştı veya üstünde: Düşey hız referansını 0 yap (Sabit kal)
        v_ref = 0.0;
    elseif z <= z_hover_start
        % Araç henüz 2 metrenin altında veya sınırda: Maksimum tırmanış hızı ver
        v_ref = v_climb;
    else
        % 2 metre ile 5 metre arasında dinamik yaklaşım (Yumuşak duruş için)
        % Hedefe yaklaştıkça hız referansını lineer olarak azaltarak sönümleme yapıyoruz
        denom_hover = z_hover_target - z_hover_start;
        if denom_hover < 1e-4, denom_hover = 1e-4; end
        
        % Hedefe olan mesafe oranı (5 metreye yaklaştıkça ratio_hover -> 0 olur)
        ratio_hover = (z_hover_target - z) / denom_hover;
        ratio_hover = max(min(ratio_hover, 1.0), 0.0);
        
        % Hız referansı (Hedefe yaklaştıkça 0'a yaklaşır, 2 metreye yaklaştıkça v_climb olur)
        v_ref = ratio_hover * v_climb;
    end
    
    % Hover modundayken de v_entry_speed'i güncel tutuyoruz ki landing moduna ani 
    % bir geçiş olursa hafıza hatalı kalmasın.
    v_entry_speed = vz;

else
    % Diğer modlar (Motor Off vb.)
    v_ref = 0.0;
    motor_status = 0.0;
    v_entry_speed = vz; % Aktif değilken hızı takip etmeye devam et
end
end
